simulink model "Teste1"  (R2025b)
settings: Solver=ode4  StartTime=0.0  StopTime=inf  FixedStep=0.010  RelTol=1e-3  EnableMultiTasking=on
undefined symbols (not defined in the file): bits
libraries: stm32blockslib x9, hdlsllib x1, stmutilitieslib x1
settings Model: STM32="{\"I2CControllerWrite\":[{\"ID\":\"untitled:20\"},{\"ID\":\"Teste1:20\"},{\"ID\":\"Teste1:70\"},{\"ID\":\"Teste1:80\"},{\"ID\":\"Teste1:180\"}],\"SPIControllerTransfer\":[{\"ID\":\"Teste1:126\"},{\"ID\":\"Teste1:160\"},{\"ID\":\"Teste1:222\"}],\"EncoderBlock\":{\"ID\":\"Teste1:108\"},\"I2CControllerRead\":{\"ID\":\"Teste1:284\"}}"  SimulationMode=external  Creator=IEE-S  LastModifiedBy=IEE-S
settings OptimizationCC: EnhancedBackFolding=on  PassReuseOutputArgsAs=Individual arguments  ZeroExternalMemoryAtStartup=off  ZeroInternalMemoryAtStartup=off  MaxStackSize=512  OptimizeBlockOrder=speed  DifferentSizesBufferReuse=on  OptimizationCustomize=off  EfficientTunableParamExpr=on
settings DebuggingCC: ParameterTunabilityLossMsg=error
settings HardwareCC: ProdBitPerPointer=32.0  ProdBitPerSizeT=32.0  ProdBitPerPtrDiffT=32.0  ProdLargestAtomicInteger=Long  ProdLargestAtomicFloat=Double  ProdWordSize=32.0  ProdLongLongMode=on  ProdHWDeviceType=ARM Compatible->ARM Cortex-M
settings SFSimCC: MATLABDynamicMemAlloc=off
settings RTWCC: SystemTargetFile=ert.tlc  HardwareBoard=STM32F4xx Based  TemplateMakefile=ert_default_tmf  Toolchain=GNU Tools for ARM Embedded Processors  Description=Embedded Coder
settings CodeAppCC: ForceParamTrailComments=on  IgnoreCustomStorageClasses=off  OperatorAnnotations=on  SimulinkDataObjDesc=on  SFDataObjDesc=on  InsertBlockDesc=on
settings ERTTargetCC: ExtModeTransport=3.0  ExtModeStaticAlloc=on  ExtModeStaticAllocSize=2048.0  ExtModeMexFile=ext_xcp  ExtModeIntrfLevel=Level2 - Open  InlinedParameterPlacement=Hierarchical  TargetLangStandard=C99 (ISO)  CodeReplacementLibrary=ARM Cortex-M  SupportContinuousTime=on

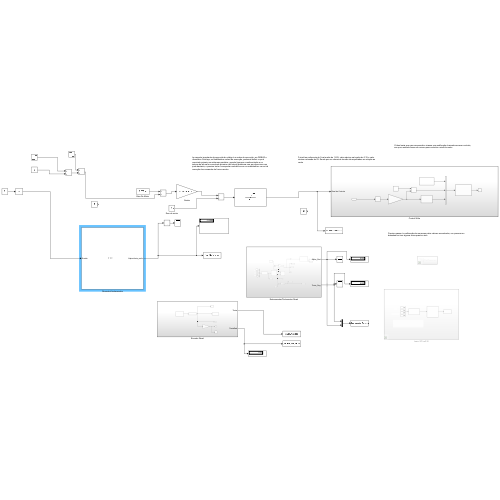
[thumbnail: Simulink's stored preview of the top-level diagram]
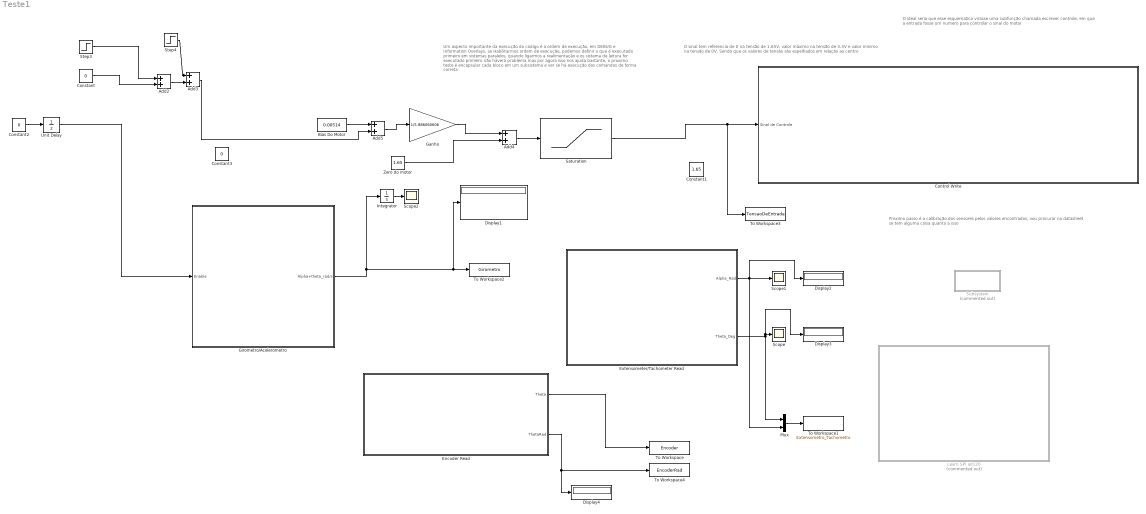
== system Teste1 ==
  note: Proximo passo é a calibração dos sensores pelos valores encontrados, vou procurar no datasheet se tem alguma coisa quanto a isso
  note: Um aspecto importante da execução do código é a ordem de execução, em DEBUG e Information Overlays, se Habilitarmos ordem de execução, podemos definir o que é executado primeiro em sistemas paralelos, quando ligarmos a realimentação e os sistema de leitura for executado primeiro não háverá problema mas por agora isso nos ajuda bastante, o proximo teste é encapsular cada bloco em um subsistema e ver se há execução dos comandos de forma correta
  note: O ideal seria que esse esquematico virasse uma subfunção chamada escrever controle, em que a entrada fosse um numero para controlar o sinal do motor
  note: O sinal tem referencia de 0 na tensão de 1.65V, valor máximo na tensão de 3.3V e valor minimo na tensão de 0V. Sendo que os valores de tensão são espelhados em relação ao centro
  Add{2..5} (4 alike) : Sum
  Bias Do Motor : Constant  Value=0.00514
  Constant : Constant  Value=0
  Constant1 : Constant  Value=1.65
  Constant2 : Constant  Value=0
  Constant3 : Constant  Value=0
  Control Write : Subsystem  Priority=6
  Display{1..4} (4 alike) : Display
  Encoder Read : Subsystem  Priority=3
  Extensometer/Tachometer Read : Subsystem  Priority=4
  Ganho : Gain  Gain=1/5.886060606
  Girometro/Acelerometro : Subsystem  Priority=1
      mask Display: image('IMU.jpg');
  Integrator : Integrator
  Learn SPI ad120 : Subsystem  Priority=4  Commented=on
  Mux : Mux  Inputs=2
  Saturation : Saturate  UpperLimit=3.3  LowerLimit=0
  Scope : Scope
      settings: ActiveDisplayYMinimum=1782.2820365229677  ActiveDisplayYMaximum=2183.0618859160627
  Scope1 : Scope
      settings: ActiveDisplayYMinimum=822.858912713687  ActiveDisplayYMaximum=3374.2054786139925  DataLoggingVariableName=ScopeData4
  Scope2 : Scope
      settings: ActiveDisplayYMinimum=29.96277740756102  ActiveDisplayYMaximum=79.082685155212445  DataLoggingVariableName=ScopeData3
  Step3 : Step  Time=2  After=1.5  SampleTime=0
  Step4 : Step  Time=2.5  After=-1.5  SampleTime=0
  Subsystem : Subsystem  Commented=on
  To Workspace : ToWorkspace  VariableName=Encoder  SaveFormat=Timeseries  SampleTime=-1
  To Workspace1 : ToWorkspace  VariableName=Extensometro_Tachometro  SaveFormat=Timeseries  SampleTime=-1
  To Workspace2 : ToWorkspace  VariableName=Girometro  SaveFormat=Timeseries  SampleTime=-1
  To Workspace3 : ToWorkspace  VariableName=TensaoDeEntrada  SaveFormat=Timeseries  SampleTime=-1
  To Workspace4 : ToWorkspace  VariableName=EncoderRad  SaveFormat=Timeseries  SampleTime=-1
  Unit Delay : UnitDelay  InitialCondition=1  SampleTime=-1  HasFrameUpgradeWarning=on
  Zero do motor : Constant  Value=1.65
  wires:
  Extensometer/Tachometer Read/2(Theta_Deg) -> Display3/1, Scope/1, Mux/1
  Extensometer/Tachometer Read/1(Alpha_Rad) -> Display2/1, Scope1/1, Mux/2
  Mux/1 -> To Workspace1/1
  Girometro/Acelerometro/1(Alpha+theta_rad/s) -> Integrator/1, Display1/1, To Workspace2/1
  Unit Delay/1 -> Girometro/Acelerometro/1(Enable)
  Encoder Read/2(ThetaRad) -> To Workspace4/1, Display4/1
  Encoder Read/1(Theta) -> To Workspace/1
  Constant2/1 -> Unit Delay/1
  Step4/1 -> Add3/1
  Add2/1 -> Add3/2
  Step3/1 -> Add2/1
  Constant/1 -> Add2/2
  Integrator/1 -> Scope2/1
  Saturation/1 -> To Workspace3/1, Control Write/1(Sinal de Controle)
  Zero do motor/1 -> Add4/2
  Bias Do Motor/1 -> Add5/1
  Add5/1 -> Ganho/1
  Ganho/1 -> Add4/1
  Add4/1 -> Saturation/1
  Add3/1 -> Add5/2

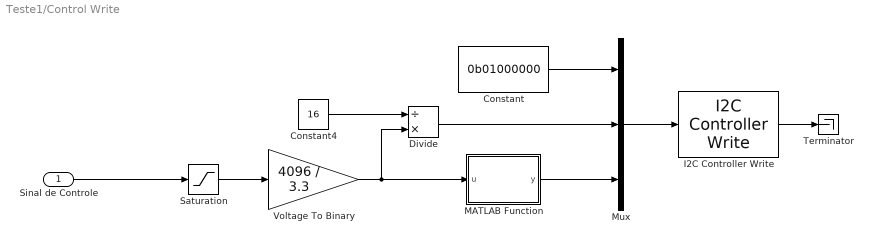
== system Teste1/Control Write ==
  Sinal de Controle : Inport
  Constant : Constant  Value=0b01000000  OutDataTypeStr=uint8
  Constant4 : Constant  Value=16
  Divide : Product  Inputs=/*  OutDataTypeStr=uint8
  I2C Controller Write : stm32blockslib/I2C Controller Write  I2CModule=I2C1  Mode=Controller  AddressingMode=7-bits  PeripheralByteOrder=BigEndian  OwnPeripheralAddress=uint8(170)  PeripheralAddressVia=Dialog  PeripheralAddress=0x60  RegisterAddressMode=off  RegisterAddressVia=Dialog  RegisterAddress=1  RepeatedStart=off  NoAck=off  OutputStatus=on  BlockMode=Transmit  DataType=uint8  DataLength=1  Timeout=0.001  SampleTime=-1
      settings: LibrarySourceBlock=stm32f4xxblockslib/I2C Controller Write
  MATLAB Function : MATLAB Function  TreatAsAtomicUnit=on
  Mux : Mux  Inputs=3
  Saturation : Saturate  UpperLimit=3.3  LowerLimit=0  OutDataTypeStr=Inherit: Inherit via back propagation
  Terminator : Terminator
  Voltage To Binary : Gain  Gain=4096 / 3.3  ParamDataTypeStr=uint16
  wires:
  Voltage To Binary/1 -> Divide/2, MATLAB Function/1(u)
  Constant4/1 -> Divide/1
  Constant/1 -> Mux/1
  Divide/1 -> Mux/2
  I2C Controller Write/1 -> Terminator/1
  MATLAB Function/1(y) -> Mux/3
  Saturation/1 -> Voltage To Binary/1
  Mux/1 -> I2C Controller Write/1
  Sinal de Controle/1 -> Saturation/1

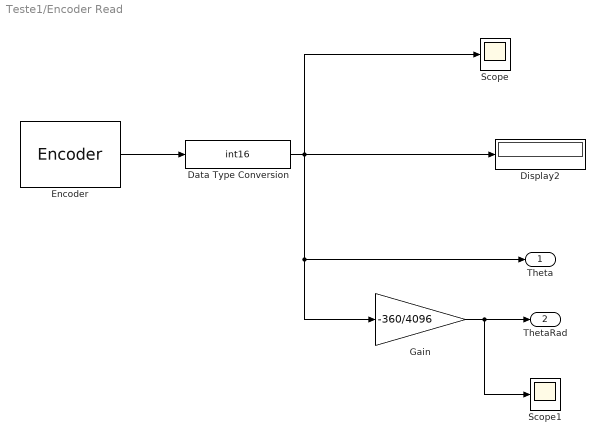
== system Teste1/Encoder Read ==
  Data Type Conversion : DataTypeConversion  OutDataTypeStr=int16  RndMeth=Round  SaturateOnIntegerOverflow=off
  Display2 : Display
  Encoder : stm32blockslib/Encoder  TimerModule=TIM4  EnableResetInput=off  OutputDirection=off  SampleTime=-1
      settings: LibrarySourceBlock=stm32f4xxblockslib/Encoder
  Gain : Gain  Gain=-360/4096
  Scope : Scope
      settings: ActiveDisplayYMinimum=-1161  ActiveDisplayYMaximum=128.99999999999997
  Scope1 : Scope
      settings: ActiveDisplayYMinimum=-12.677807615034702  ActiveDisplayYMaximum=73.709890997310026  DataLoggingVariableName=ScopeData7
  Theta : Outport
  ThetaRad : Outport  Port=2
  wires:
  Encoder/1 -> Data Type Conversion/1
  Data Type Conversion/1 -> Scope/1, Theta/1, Gain/1, Display2/1
  Gain/1 -> Scope1/1, ThetaRad/1

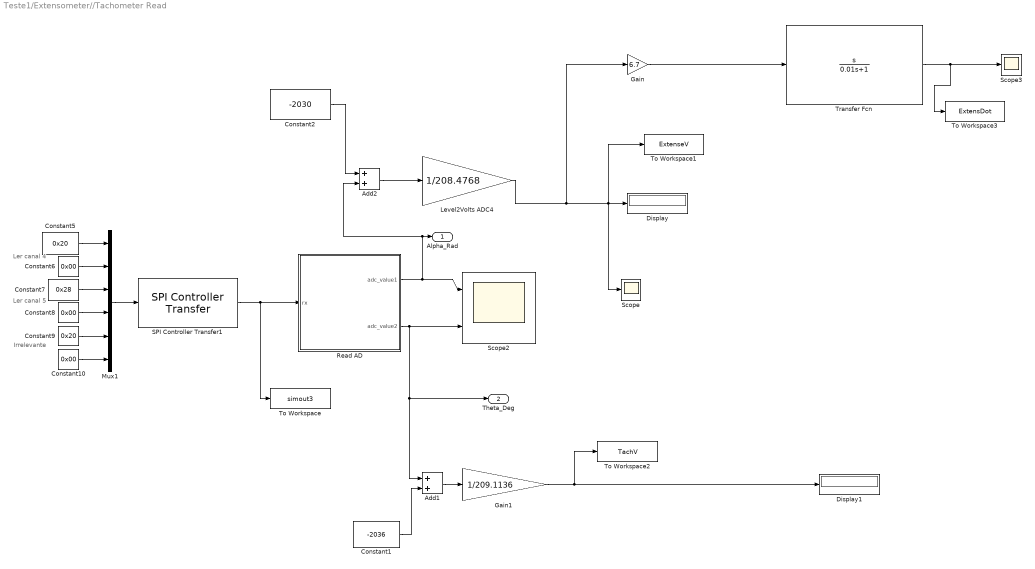
== system Teste1/Extensometer//Tachometer Read ==
  note: Irrelevante
  note: Ler canal 5
  note: Ler canal 4
  Add1 : Sum
  Add2 : Sum
  Constant1 : Constant  Value=-2036
  Constant10 : Constant  Value=0x00  OutDataTypeStr=uint8
  Constant2 : Constant  Value=-2030
  Constant5 : Constant  Value=0x20  OutDataTypeStr=uint8
  Constant6 : Constant  Value=0x00  OutDataTypeStr=uint8
  Constant7 : Constant  Value=0x28  OutDataTypeStr=uint8
  Constant8 : Constant  Value=0x00  OutDataTypeStr=uint8
  Constant9 : Constant  Value=0x20  OutDataTypeStr=uint8
  Display : Display
  Display1 : Display
  Gain : Gain  Gain=6.7
  Gain1 : Gain  Gain=1/209.1136
  Level2Volts ADC4 : Gain  Gain=1/208.4768
  Mux1 : Mux  Inputs=6
  Read AD : MATLAB Function  TreatAsAtomicUnit=on
  SPI Controller Transfer1 : stm32blockslib/SPI Controller Transfer  SPIModuleSelect=SPI2  ClockPolarity=Low  ClockPhase=1 Edge  SPIModule=uint32(0)  Mode=Master  BusSpeed=uint32(1000000)  FirstBitToTransfer=Most significant bit (MSB)  ClockMode=0  BlockFunction=Transfer  EnableRegisterAddress=off  RegisterAddress=0  OutputDataType=uint8  OutputDataLength=1  OutputStatus=off  BlockingMode=on  Timeout=1  DataBits=8  UseCustomSSPin=Explicit GPIO calls  ActiveLowSSPin=Active low  Port_Select=GPIOA  Pin=4
      settings: LibrarySourceBlock=stm32f4xxblockslib/SPI Controller Transfer
  Scope : Scope
      settings: ActiveDisplayYMinimum=-0.40783945168836933  ActiveDisplayYMaximum=0.49149339441480261  DataLoggingVariableName=ScopeData6
  Scope2 : Scope  NumInputPorts=2
      settings: ActiveDisplayYMinimum=840.43616748858926  ActiveDisplayYMaximum=3838.9026152924334  DataLoggingVariableName=ScopeData2
  Scope3 : Scope
      settings: ActiveDisplayYMinimum=-133.85888820809296  ActiveDisplayYMaximum=147.146193579922  DataLoggingVariableName=ScopeData8
  To Workspace : ToWorkspace  VariableName=simout3  SaveFormat=Timeseries  SampleTime=-1
  To Workspace1 : ToWorkspace  VariableName=ExtenseV  SaveFormat=Timeseries  SampleTime=-1
  To Workspace2 : ToWorkspace  VariableName=TachV  SaveFormat=Timeseries  SampleTime=-1
  To Workspace3 : ToWorkspace  VariableName=ExtensDot  SaveFormat=Timeseries  SampleTime=-1
  Transfer Fcn : TransferFcn  Numerator=[1 0]  Denominator=[0.01 1]
  Alpha_Rad : Outport
  Theta_Deg : Outport  Port=2
  wires:
  Mux1/1 -> SPI Controller Transfer1/1
  SPI Controller Transfer1/1 -> To Workspace/1, Read AD/1(rx)
  Constant5/1 -> Mux1/1
  Constant6/1 -> Mux1/2
  Constant7/1 -> Mux1/3
  Constant8/1 -> Mux1/4
  Constant9/1 -> Mux1/5
  Constant10/1 -> Mux1/6
  Read AD/2(adc_value2) -> Scope2/2, Add1/1, Theta_Deg/1
  Add1/1 -> Gain1/1
  Gain1/1 -> Display1/1, To Workspace2/1
  Constant1/1 -> Add1/2
  Add2/1 -> Level2Volts ADC4/1
  Read AD/1(adc_value1) -> Scope2/1, Add2/2, Alpha_Rad/1
  Constant2/1 -> Add2/1
  Level2Volts ADC4/1 -> Gain/1, Display/1, Scope/1, To Workspace1/1
  Transfer Fcn/1 -> To Workspace3/1, Scope3/1
  Gain/1 -> Transfer Fcn/1

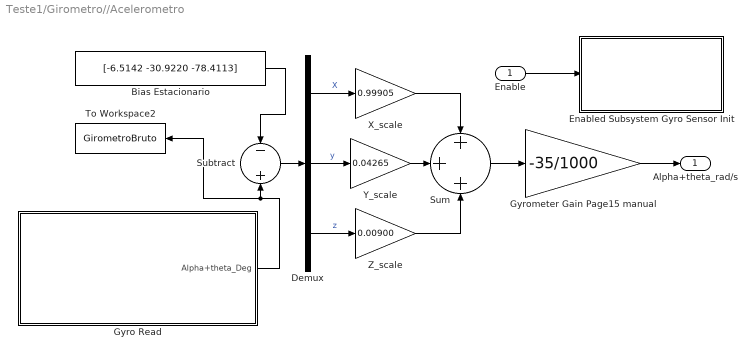
== system Teste1/Girometro//Acelerometro ==
  Enable : Inport
  Bias Estacionario : Constant  Value=[-6.5142 -30.9220 -78.4113]
  Demux : Demux  Outputs=3
  Enabled Subsystem Gyro Sensor Init : Subsystem  Priority=1  TreatAsAtomicUnit=on
  Gyro Read : Subsystem  Priority=2
  Gyrometer Gain Page15 manual : Gain  Gain=-35/1000
  Subtract : Sum  Inputs=-+
  Sum : Sum  Inputs=+++
  To Workspace2 : ToWorkspace  VariableName=GirometroBruto  SaveFormat=Timeseries  SampleTime=-1
  X_scale : Gain  Gain=0.99905
  Y_scale : Gain  Gain=0.04265
  Z_scale : Gain  Gain=0.00900
  Alpha+theta_rad/s : Outport
  wires:
  Enable/1 -> Enabled Subsystem Gyro Sensor Init/Enable
  Demux/3 -> Z_scale/1  "z"
  Demux/1 -> X_scale/1  "X"
  Gyrometer Gain Page15 manual/1 -> Alpha+theta_rad/s/1
  Y_scale/1 -> Sum/2
  Sum/1 -> Gyrometer Gain Page15 manual/1
  Z_scale/1 -> Sum/3
  X_scale/1 -> Sum/1
  Demux/2 -> Y_scale/1  "y"
  Bias Estacionario/1 -> Subtract/1
  Subtract/1 -> Demux/1
  Gyro Read/1(Alpha+theta_Deg) -> To Workspace2/1, Subtract/2

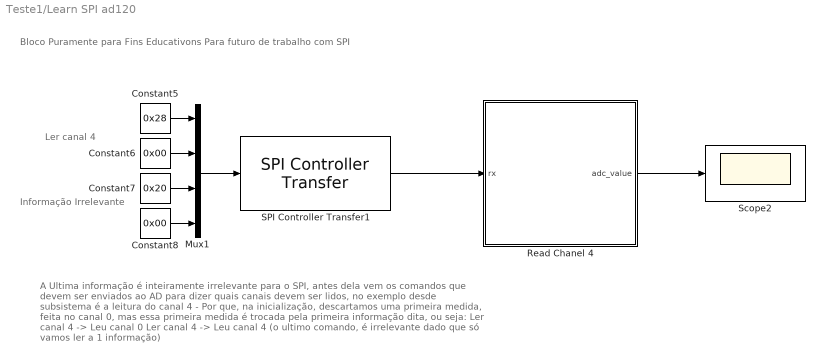
== system Teste1/Learn SPI ad120 ==
  note: A Ultima informação é inteiramente irrelevante para o SPI, antes dela vem os comandos que devem ser enviados ao AD para dizer quais canais devem ser lidos, no exemplo desde subsistema é a leitura do canal 4 - Por que, na inicialização, descartamos uma primeira medida, feita no canal 0, mas essa primeira medida é trocada pela primeira informação dita, ou seja:
      | Ler canal 4 -> Leu canal 0
      | Ler canal 4 -> Leu canal 4 (o ultimo comando, é irrelevante dado que só vamos ler a 1 informação)
  note: Bloco Puramente para Fins Educativons Para futuro de trabalho com SPI
  note: Informação Irrelevante
  note: Ler canal 4
  Constant5 : Constant  Value=0x28  OutDataTypeStr=uint8
  Constant6 : Constant  Value=0x00  OutDataTypeStr=uint8
  Constant7 : Constant  Value=0x20  OutDataTypeStr=uint8
  Constant8 : Constant  Value=0x00  OutDataTypeStr=uint8
  Mux1 : Mux
  Read Chanel 4 : MATLAB Function  TreatAsAtomicUnit=on
  SPI Controller Transfer1 : stm32blockslib/SPI Controller Transfer  SPIModuleSelect=SPI2  ClockPolarity=Low  ClockPhase=1 Edge  SPIModule=uint32(0)  Mode=Master  BusSpeed=uint32(1000000)  FirstBitToTransfer=Most significant bit (MSB)  ClockMode=0  BlockFunction=Transfer  EnableRegisterAddress=off  RegisterAddress=0  OutputDataType=uint8  OutputDataLength=1  OutputStatus=off  BlockingMode=on  Timeout=0.001  DataBits=8  UseCustomSSPin=Explicit GPIO calls  ActiveLowSSPin=Active low  Port_Select=GPIOA  Pin=5
      settings: LibrarySourceBlock=stm32f4xxblockslib/SPI Controller Transfer
  Scope2 : Scope
      settings: ActiveDisplayYMinimum=342.18345535588639  ActiveDisplayYMaximum=5853.6707282673206  DataLoggingVariableName=ScopeData2
  wires:
  Read Chanel 4/1(adc_value) -> Scope2/1
  Constant6/1 -> Mux1/2
  SPI Controller Transfer1/1 -> Read Chanel 4/1(rx)
  Mux1/1 -> SPI Controller Transfer1/1
  Constant5/1 -> Mux1/1
  Constant7/1 -> Mux1/3
  Constant8/1 -> Mux1/4

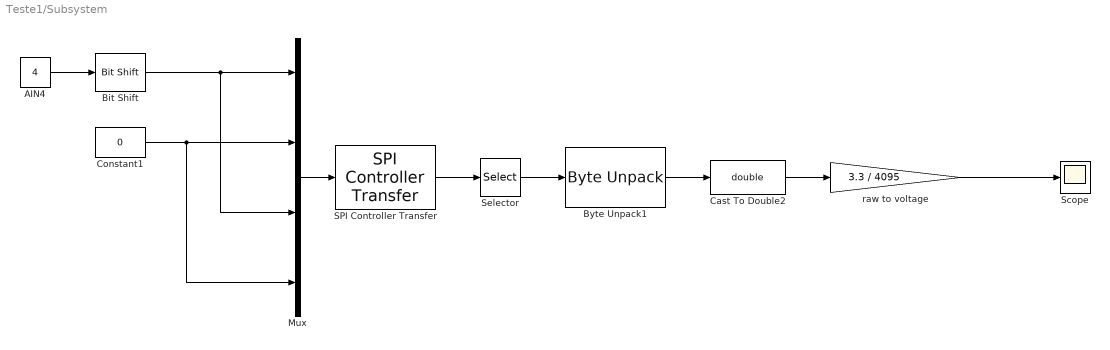
== system Teste1/Subsystem ==
  AIN4 : Constant  Value=4  OutDataTypeStr=uint8
  Bit Shift : hdlsllib/Logic and Bit Operations/Bit Shift  mode=Shift Left Logical  N=3
  Byte Unpack1 : stmutilitieslib/Byte Unpack  dimensions={1}  datatypes={'uint16'}  byteAlign=2  blockPlatform=stm32f4discovery
  Cast To Double2 : DataTypeConversion  OutDataTypeStr=double  SaturateOnIntegerOverflow=off  RndMeth=Floor
  Constant1 : Constant  Value=0  OutDataTypeStr=uint8
  Mux : Mux
  SPI Controller Transfer : stm32blockslib/SPI Controller Transfer  SPIModuleSelect=SPI2  ClockPolarity=Low  ClockPhase=1 Edge  SPIModule=uint32(0)  Mode=Master  BusSpeed=uint32(1000000)  FirstBitToTransfer=Most significant bit (MSB)  ClockMode=0  BlockFunction=Transfer  EnableRegisterAddress=off  RegisterAddress=0  OutputDataType=uint8  OutputDataLength=1  OutputStatus=off  BlockingMode=on  Timeout=1  DataBits=8  UseCustomSSPin=Explicit GPIO calls  ActiveLowSSPin=Active low  Port_Select=GPIOA  Pin=4
      settings: LibrarySourceBlock=stm32f4xxblockslib/SPI Controller Transfer
  Scope : Scope
      settings: ActiveDisplayYMinimum=-0.44059876699767653  ActiveDisplayYMaximum=4.9466368983020628  DataLoggingVariableName=ScopeData5
  Selector : Selector  InputPortWidth=4  IndexOptions=Index vector (dialog)  Indices=[4 3]  OutputSizes=1
  raw to voltage : Gain  Gain=3.3 / 4095
  wires:
  Cast To Double2/1 -> raw to voltage/1
  Bit Shift/1 -> Mux/1, Mux/3
  Constant1/1 -> Mux/2, Mux/4
  Selector/1 -> Byte Unpack1/1
  SPI Controller Transfer/1 -> Selector/1
  AIN4/1 -> Bit Shift/1
  Mux/1 -> SPI Controller Transfer/1
  Byte Unpack1/1 -> Cast To Double2/1
  raw to voltage/1 -> Scope/1

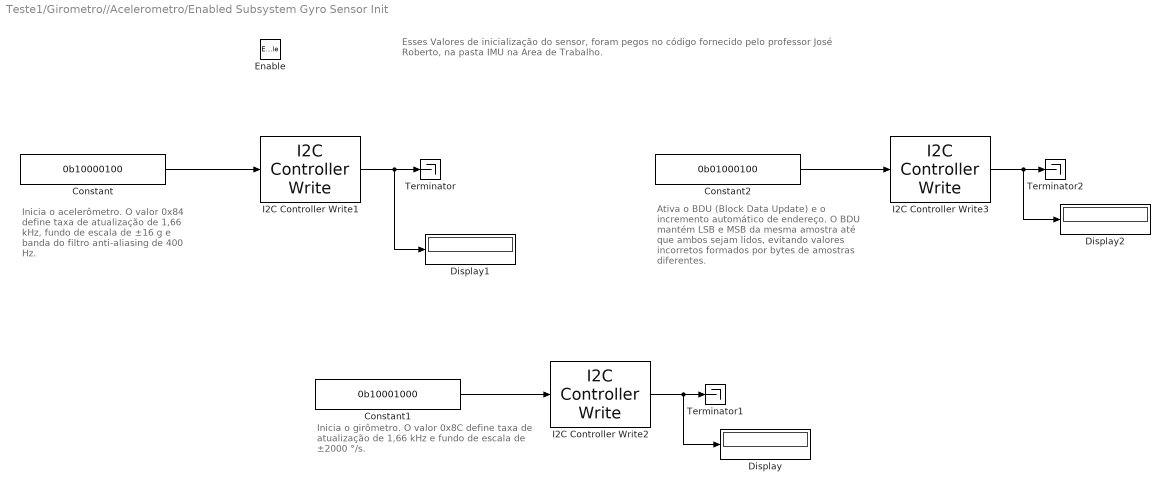
== system Teste1/Girometro//Acelerometro/Enabled Subsystem Gyro Sensor Init ==
  note: Inicia o acelerômetro. O valor 0x84 define taxa de atualização
      | de 1,66 kHz, fundo de escala de ±16 g e banda do filtro anti-aliasing de 400 Hz.
  note: Inicia o girômetro. O valor 0x8C define taxa de atualização
      | de 1,66 kHz e fundo de escala de ±2000 °/s.
  note: Ativa o BDU (Block Data Update) e o incremento automático de endereço.
      | O BDU mantém LSB e MSB da mesma amostra até que ambos sejam lidos,
      | evitando valores incorretos formados por bytes de amostras diferentes.
  note: Esses Valores de inicialização do sensor, foram pegos no código fornecido pelo professor José Roberto, na pasta IMU na Area de Trabalho.
  Enable : EnablePort
  Constant : Constant  Value=0b10000100
  Constant1 : Constant  Value=0b10001000
  Constant2 : Constant  Value=0b01000100
  Display : Display
  Display1 : Display
  Display2 : Display
  I2C Controller Write1 : stm32blockslib/I2C Controller Write  I2CModule=I2C1  Mode=Controller  AddressingMode=7-bits  PeripheralByteOrder=BigEndian  OwnPeripheralAddress=uint8(170)  PeripheralAddressVia=Dialog  PeripheralAddress=0b1101010  RegisterAddressMode=on  RegisterAddressVia=Dialog  RegisterAddress=0x10  RepeatedStart=off  NoAck=off  OutputStatus=on  BlockMode=Transmit  DataType=uint8  DataLength=1  Timeout=0.001  SampleTime=-1
      settings: LibrarySourceBlock=stm32f4xxblockslib/I2C Controller Write
  I2C Controller Write2 : stm32blockslib/I2C Controller Write  I2CModule=I2C1  Mode=Controller  AddressingMode=7-bits  PeripheralByteOrder=BigEndian  OwnPeripheralAddress=uint8(170)  PeripheralAddressVia=Dialog  PeripheralAddress=0b1101010  RegisterAddressMode=on  RegisterAddressVia=Dialog  RegisterAddress=0x11  RepeatedStart=off  NoAck=off  OutputStatus=on  BlockMode=Transmit  DataType=uint8  DataLength=1  Timeout=0.001  SampleTime=-1
      settings: LibrarySourceBlock=stm32f4xxblockslib/I2C Controller Write
  I2C Controller Write3 : stm32blockslib/I2C Controller Write  I2CModule=I2C1  Mode=Controller  AddressingMode=7-bits  PeripheralByteOrder=BigEndian  OwnPeripheralAddress=uint8(170)  PeripheralAddressVia=Dialog  PeripheralAddress=0x6A  RegisterAddressMode=on  RegisterAddressVia=Dialog  RegisterAddress=0x12  RepeatedStart=off  NoAck=off  OutputStatus=on  BlockMode=Transmit  DataType=uint8  DataLength=1  Timeout=0.001  SampleTime=-1
      settings: LibrarySourceBlock=stm32f4xxblockslib/I2C Controller Write
  Terminator : Terminator
  Terminator1 : Terminator
  Terminator2 : Terminator
  wires:
  Constant/1 -> I2C Controller Write1/1
  I2C Controller Write1/1 -> Display1/1, Terminator/1
  I2C Controller Write2/1 -> Display/1, Terminator1/1
  Constant1/1 -> I2C Controller Write2/1
  Constant2/1 -> I2C Controller Write3/1
  I2C Controller Write3/1 -> Terminator2/1, Display2/1

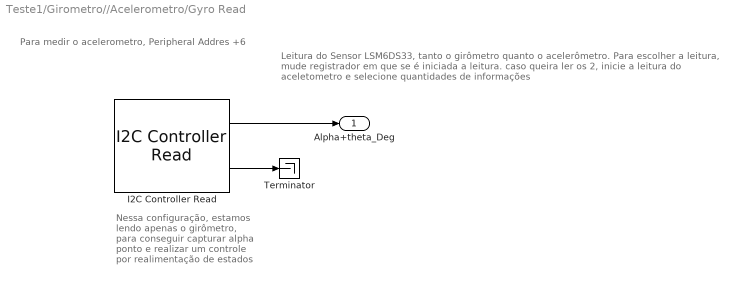
== system Teste1/Girometro//Acelerometro/Gyro Read ==
  note: Para medir o acelerometro, Peripheral Addres +6
  note: Nessa configuração, estamos lendo apenas o girômetro, para conseguir capturar alpha ponto e realizar um controle por realimentação de estados
  note: Leitura do Sensor LSM6DS33, tanto o girômetro quanto o acelerômetro. Para escolher a leitura, mude registrador em que se é iniciada a leitura. caso queira ler os 2, inicie a leitura do aceletometro e selecione quantidades de informações
  I2C Controller Read : stm32blockslib/I2C Controller Read  I2CModule=I2C1  Mode=Controller  AddressingMode=7-bits  PeripheralByteOrder=LittleEndian  OwnPeripheralAddress=uint8(170)  PeripheralAddressVia=Dialog  PeripheralAddress=0b1101010  RegisterAddressMode=on  RegisterAddressVia=Dialog  RegisterAddress=0x22  RepeatedStart=off  NoAck=off  OutputStatus=on  BlockMode=Receive  DataType=int16  DataLength=3  Timeout=0.010  SampleTime=-1
      settings: LibrarySourceBlock=stm32f4xxblockslib/I2C Controller Read
  Terminator : Terminator
  Alpha+theta_Deg : Outport
  wires:
  I2C Controller Read/1 -> Alpha+theta_Deg/1
  I2C Controller Read/2 -> Terminator/1

== matlab function Teste1/Control Write/MATLAB Function ==
  data: u input; y output
function y = fcn(u)

y = bitshift(bitand(u, uint8(15)), 4);

== matlab function Teste1/Extensometer//Tachometer Read/Read AD ==
  data: rx input; adc_value1 output; adc_value2 output
function [adc_value1, adc_value2] = decode_adc120(rx)

% Valor 1: bytes 3 e 4
raw1 = bitor(bitshift(uint16(rx(3)),8), uint16(rx(4)));
adc_value1 = bitand(raw1, hex2dec('0FFF'));

% Valor 2: bytes 5 e 6
raw2 = bitor(bitshift(uint16(rx(5)),8), uint16(rx(6)));
adc_value2 = bitand(raw2, hex2dec('0FFF'));

end

== matlab function Teste1/Learn SPI ad120/Read Chanel 4 ==
  data: rx input; adc_value output
function adc_value = decode_adc120(rx)

% rx(1) = byte alto
% rx(2) = byte baixo

raw = bitor(bitshift(uint16(rx(3)),8), uint16(rx(4)));

adc_value = bitand(raw, hex2dec('0FFF'));

end
